simulink model "Manipulator2dof_SimMdl"  (R2026a)
settings: Solver=ode15s  StopTime=20  MaxStep=0.01
values from neighbouring files (symbols this model uses):
  d = 0.2    [Manipulator2dof_SimMdl_ini.m]
  T = 0.01    [Manipulator2dof_SimMdl_ini.m]
undefined symbols (not defined in the file or in its folder): l1, manip, X, Y, Z
libraries: sm_lib x16, nesl_utility x11, SignalEditorBlockLib x1
settings Model: Creator=Bender  LastModifiedBy=natte
settings SimscapeCC: SimscapeNominalValues="[{\"value\":\"1\",\"unit\":\"A\"},{\"value\":\"1\",\"unit\":\"bar\"},{\"value\":\"1\",\"unit\":\"cm^2\"},{\"value\":\"1\",\"unit\":\"cm^3/s\"},{\"value\":\"1\",\"unit\":\"kJ/kg\"},{\"value\":\"1\",\"unit\":\"kW\"},{\"value\":\"1\",\"unit\":\"l\"},{\"value\":\"1\",\"unit\":\"N\"},{\"value\":\"1\",\"unit\":\"N*m\"},{\"value\":\"1\",\"unit\":\"V\"}]"  SimscapeLogType=none  SimscapeLogDataHistory=5000.0

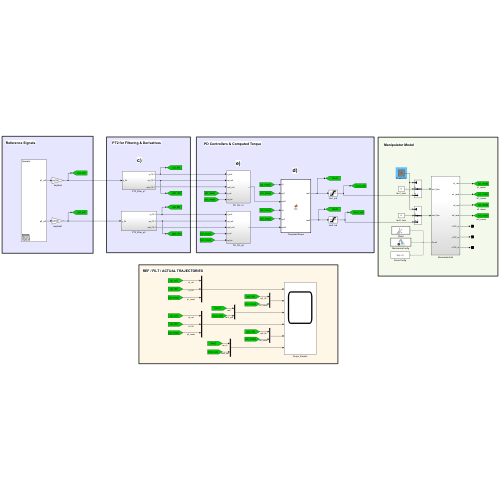
[thumbnail: Simulink's stored preview of the top-level diagram]
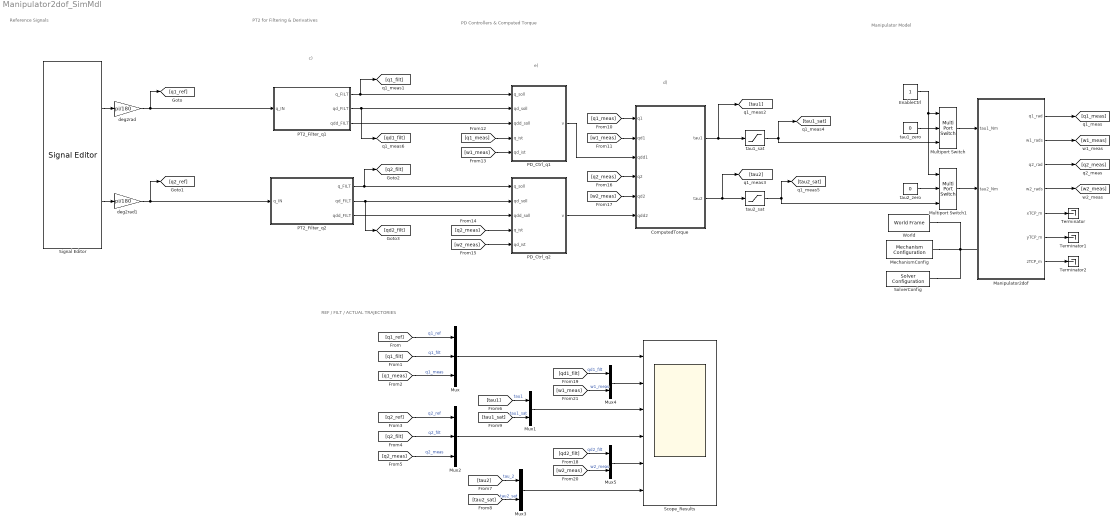
== system Manipulator2dof_SimMdl ==
  note: Reference Signals
  note: PT2 for Filtering & Derivatives
  note: PD Controllers & Computed Torque
  note: Manipulator Model
  note: REF / FILT / ACTUAL TRAJECTORIES
  note: d)
  note: c)
  note: e)
  ComputedTorque : MATLAB Function  TreatAsAtomicUnit=on
  EnableCtrl : Constant
  Manipulator2dof : Subsystem
  MechanismConfig : sm_lib/Utilities/Mechanism Configuration  UniformGravity=Constant  GravityVector=[0 0 -manip.g]  GravityVectorUnits=m/s^2  LinearizationDelta=0.001  JointModeTransitionNonlinearIterations=2
  Multiport Switch : MultiPortSwitch  DataPortOrder=Zero-based contiguous  Inputs=2  zeroidx=on  SaturateOnIntegerOverflow=off  InputSameDT=off
  Multiport Switch1 : MultiPortSwitch  DataPortOrder=Zero-based contiguous  Inputs=2  zeroidx=on  SaturateOnIntegerOverflow=off  InputSameDT=off
  Mux : Mux  Inputs=3
  Mux{1,3..5} (4 alike) : Mux  Inputs=2
  Mux2 : Mux  Inputs=3
  PD_Ctrl_q1 : Subsystem
  PD_Ctrl_q2 : Subsystem
  PT2_Filter_q1 : Subsystem
  PT2_Filter_q2 : Subsystem
  Scope_Results : Scope  NumInputPorts=6
      settings: ActiveDisplayYMinimum=-1  ActiveDisplayYMaximum=1
  Signal Editor : SignalEditorBlockLib/Signal Editor  FileName=Manipulator2dof_refSig.mat  ActiveScenario=Scenario  ActiveSignal=q1_ref  IsBus=off  OutputBusObjectStr=Bus: BusObject  SampleTime=0  ZeroCross=off  OutputAfterFinalValue=Setting to zero  Unit=inherit  PreserveSignalName=on  ApplySigPropsToAllScenarios=on  ApplySigPropsToAllSignals=off  SignalPropertySource=Dialog parameters
  SolverConfig : nesl_utility/Solver Configuration  PhysicalDomain=network_engine_domain  SubClassName=solver  LeftPortType=input  RightPortType=generic  Tones=[]  Harmonics=[]  SimulateNoise=off  Profile=off  UseLocalSampling=off  EnableSwitchedLinearOptims=on  FrequencyDomain=off  UseCCode=off  RelTol=0.001  AbsTol=0.001  MinStep=1e-09  ToWorkspace=off  RevertToSquareIcSolve=off  NumHomotopyIterations=100  PhasorMode=off  PhasorModeNumHarmonics=1  ConsistencySolver=NEWTON_XTOL_AFTER_FTOL  CanonicalOrdering=UNORDERED  OptimizeIntermediates=UNOPTIMIZED  IndexReductionMethod=DerivativeReplacement  DoDC=off  ResidualTolerance=1e-09  ConsistencyTolSource=GLOBAL  ConsistencyAbsTol=0.001  ConsistencyRelTol=0.001  ConsistencyTolFactor=0.001  UseLocalSolver=off  LocalSolverChoice=NE_BACKWARD_EULER_ADVANCER  ResolveIndetEquations=on  FunctionEvalNumThread=1  LocalSolverSampleTime=0.001  DoFixedCost=off  MaxNonlinIter=3  MaxModeIter=2  ComputeImpulses=off  ImpulseIterations=2  LinearAlgebra=auto  LinearAlgebraNumThread=0  EquationFormulation=NE_TIME_EF  DelaysMemoryBudget=1024  AutomaticFiltering=on  FilteringTimeConstant=0.001  PartitionStorageMethod=AS_NEEDED  PartitionMemoryBudget=1024  PartitionMethod=ROBUST  MultibodyUseLocalSolver=off  MultibodyLocalSolverChoice=ODE1  MultibodyLocalSolverSampleTime=0.001
  Terminator : Terminator
  Terminator1 : Terminator
  Terminator2 : Terminator
  World : sm_lib/Frames and Transforms/World Frame
  deg2rad : Gain  Gain=pi/180
  deg2rad1 : Gain  Gain=pi/180
  tau1_sat : Saturate  UpperLimit=manip.tau1_max  LowerLimit=-manip.tau1_max
  tau1_zero : Constant  Value=0
  tau2_sat : Saturate  UpperLimit=manip.tau2_max  LowerLimit=-manip.tau2_max
  tau2_zero : Constant  Value=0
  wires:
  Manipulator2dof/1(q1_rad) -> [q1_meas]
  Manipulator2dof/3(q2_rad) -> [q2_meas]
  Manipulator2dof/4(w2_rads) -> [w2_meas]
  tau1_sat/1 -> [tau1_sat], Multiport Switch/3
  Manipulator2dof/2(w1_rads) -> [w1_meas]
  tau2_sat/1 -> [tau2_sat], Multiport Switch1/3
  Mux/1 -> Scope_Results/1
  Signal Editor/1 -> deg2rad/1
  PT2_Filter_q1/1(q_FILT) -> [q1_filt], PD_Ctrl_q1/1(q_soll)
  PT2_Filter_q1/2(qd_FILT) -> [qd1_filt], PD_Ctrl_q1/2(qd_soll)
  PT2_Filter_q1/3(qdd_FILT) -> PD_Ctrl_q1/3(qdd_soll)
  deg2rad/1 -> PT2_Filter_q1/1(q_IN), [q1_ref]
  Signal Editor/2 -> deg2rad1/1
  Mux1/1 -> Scope_Results/3
  PT2_Filter_q2/1(q_FILT) -> PD_Ctrl_q2/1(q_soll), [q2_filt]
  PT2_Filter_q2/2(qd_FILT) -> [qd2_filt], PD_Ctrl_q2/2(qd_soll)
  PT2_Filter_q2/3(qdd_FILT) -> PD_Ctrl_q2/3(qdd_soll)
  deg2rad1/1 -> PT2_Filter_q2/1(q_IN), [q2_ref]
  Mux2/1 -> Scope_Results/4
  Mux3/1 -> Scope_Results/6
  [q1_meas] -> Mux/3  "q1_meas"
  [q1_filt] -> Mux/2  "q1_filt"
  [q1_ref] -> Mux/1  "q1_ref"
  [q2_ref] -> Mux2/1  "q2_ref"
  [q2_filt] -> Mux2/2  "q2_filt"
  [q2_meas] -> Mux2/3  "q2_meas"
  [tau1] -> Mux1/1  "tau1"
  [tau2] -> Mux3/1  "tau_2"
  [tau2_sat] -> Mux3/2  "tau2_sat"
  [tau1_sat] -> Mux1/2  "tau1_sat"
  ComputedTorque/1(tau1) -> tau1_sat/1, [tau1]
  ComputedTorque/2(tau2) -> tau2_sat/1, [tau2]
  PD_Ctrl_q1/1(v) -> ComputedTorque/3(qdd1)
  [q1_meas] -> ComputedTorque/1(q1)
  [w1_meas] -> ComputedTorque/2(qd1)
  [q1_meas] -> PD_Ctrl_q1/4(q_ist)
  [w1_meas] -> PD_Ctrl_q1/5(qd_ist)
  [q2_meas] -> PD_Ctrl_q2/4(q_ist)
  [w2_meas] -> PD_Ctrl_q2/5(qd_ist)
  PD_Ctrl_q2/1(v) -> ComputedTorque/6(qdd2)
  [q2_meas] -> ComputedTorque/4(q2)
  [w2_meas] -> ComputedTorque/5(qd2)
  Mux4/1 -> Scope_Results/2
  [qd1_filt] -> Mux4/1  "qd1_filt"
  Mux5/1 -> Scope_Results/5
  [qd2_filt] -> Mux5/1  "qd2_filt"
  [w2_meas] -> Mux5/2  "w2_meas"
  [w1_meas] -> Mux4/2  "w1_meas"
  Multiport Switch/1 -> Manipulator2dof/1(tau1_Nm)
  Multiport Switch1/1 -> Manipulator2dof/2(tau2_Nm)
  EnableCtrl/1 -> Multiport Switch1/1, Multiport Switch/1
  tau1_zero/1 -> Multiport Switch/2
  tau2_zero/1 -> Multiport Switch1/2
  Manipulator2dof/5(xTCP_m) -> Terminator/1
  Manipulator2dof/6(yTCP_m) -> Terminator1/1
  Manipulator2dof/7(zTCP_m) -> Terminator2/1
  connections:
  World/RConn1 -- MechanismConfig/RConn1 -- SolverConfig/RConn1 -- Manipulator2dof/LConn1

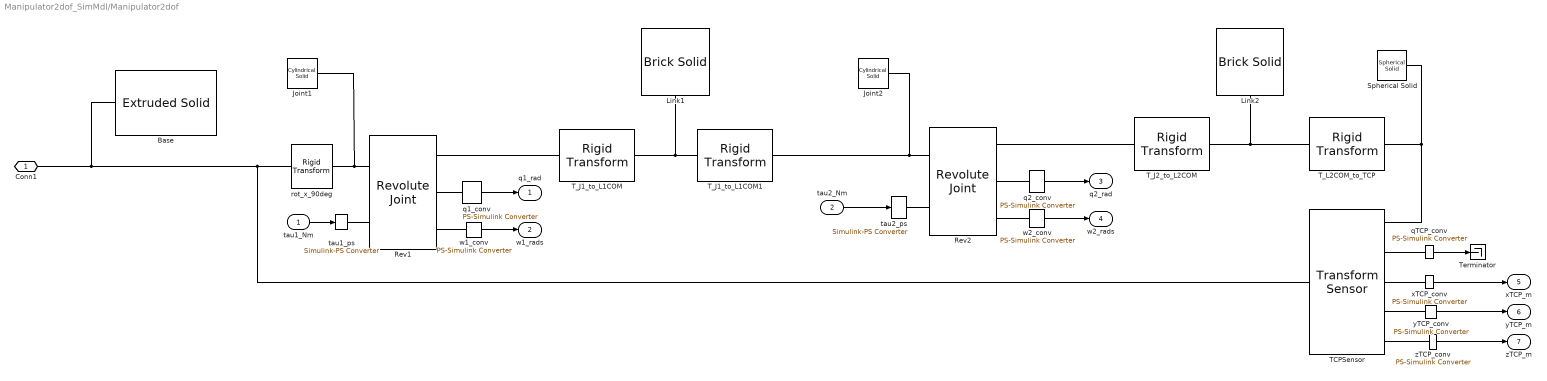
== system Manipulator2dof_SimMdl/Manipulator2dof ==
  tau1_Nm : Inport
  tau2_Nm : Inport  Port=2
  Base : sm_lib/Body Elements/Extruded Solid  ExtrusionType=Regular  PolygonNumSides=3  PolygonOuterRadius=0.2  PolygonOuterRadiusUnits=m  ExportEntireGeometry=off  ExtrusionCrossSection=[1 1; -1 1; -1 -1; 1 -1]  ExtrusionCrossSectionUnits=m  ExportConvexHullGeometry=off  ExtrusionLength=0.05  ExtrusionLengthUnits=m  InertiaType=PointMass  BasedOnType=Density  Density=1000  DensityUnits=kg/(m^3)  Mass=20  MassUnits=kg  CenterOfMass=[0 0 0]  CenterOfMassUnits=m  MomentsOfInertia=[10000 10000 10000]  MomentsOfInertiaUnits=kg*m^2  ProductsOfInertia=[10000 10000 10000]  ProductsOfInertiaUnits=kg*m^2  GraphicType=FromGeometry  MarkerShape=Sphere  MarkerSize=10  GraphicVisPropType=SimpleVisualProperties  GraphicDiffuseColor=[0.2 0.2 0.2]  GraphicOpacity=1  GraphicSpecularColor=[0.5 0.5 0.5 1.0]  GraphicAmbientColor=[0.15 0.15 0.15 1.0]  GraphicEmissiveColor=[0.0 0.0 0.0 1.0]  GraphicShininess=0  DoExposeReferenceFrame=off  SerializedFrames=<Frames><Frame><Id>Frame1</Id><Value><Name>F1</Name><Origin><Source>GeometricFeature</Source><FeatureName>side curve 2</FeatureName></Origin><PrimaryAxis><DefinedDirection>-Z</DefinedDirection><Source>GeometricFeature</Source><SourceDirection>+Z</SourceDirection><FeatureName>side surface 3</FeatureName></PrimaryAxis><SecondaryAxis><DefinedDirection>+X</DefinedDirection><Source>ReferenceFrame</Source><SourceDirection>+X</SourceDirection><FeatureName></FeatureName></SecondaryAxis></Value></Frame></Frames>
  Joint1 : sm_lib/Body Elements/Cylindrical Solid  CylinderRadius=0.05  CylinderRadiusUnits=m  CylinderLength=0.05  CylinderLengthUnits=m  ExportEntireGeometry=off  InertiaType=PointMass  BasedOnType=Density  Density=1000  DensityUnits=kg/m^3  Mass=0  MassUnits=kg  CenterOfMass=[0 0 0]  CenterOfMassUnits=m  MomentsOfInertia=[1 1 1]  MomentsOfInertiaUnits=kg*m^2  ProductsOfInertia=[0 0 0]  ProductsOfInertiaUnits=kg*m^2  GraphicType=FromGeometry  MarkerShape=Sphere  MarkerSize=10  GraphicVisPropType=SimpleVisualProperties  GraphicDiffuseColor=[0.7216 0.7216 0.7216]  GraphicOpacity=1  GraphicSpecularColor=[0.5 0.5 0.5 1.0]  GraphicAmbientColor=[0.15 0.15 0.15 1.0]  GraphicEmissiveColor=[0.0 0.0 0.0 1.0]  GraphicShininess=75  DoExposeReferenceFrame=on  SerializedFrames=<Frames/>
  Joint2 : sm_lib/Body Elements/Cylindrical Solid  CylinderRadius=0.05  CylinderRadiusUnits=m  CylinderLength=0.05  CylinderLengthUnits=m  ExportEntireGeometry=off  InertiaType=PointMass  BasedOnType=Density  Density=1000  DensityUnits=kg/m^3  Mass=manip.m1plant  MassUnits=kg  CenterOfMass=[0 0 0]  CenterOfMassUnits=m  MomentsOfInertia=[1 1 1]  MomentsOfInertiaUnits=kg*m^2  ProductsOfInertia=[0 0 0]  ProductsOfInertiaUnits=kg*m^2  GraphicType=FromGeometry  MarkerShape=Sphere  MarkerSize=10  GraphicVisPropType=SimpleVisualProperties  GraphicDiffuseColor=[0.7216 0.7216 0.7216]  GraphicOpacity=1  GraphicSpecularColor=[0.5 0.5 0.5 1.0]  GraphicAmbientColor=[0.15 0.15 0.15 1.0]  GraphicEmissiveColor=[0.0 0.0 0.0 1.0]  GraphicShininess=75  DoExposeReferenceFrame=on  SerializedFrames=<Frames/>
  Link1 : sm_lib/Body Elements/Brick Solid  BrickDimensions=[manip.l1 manip.linkWidth manip.linkThickness]  BrickDimensionsUnits=m  ExportEntireGeometry=off  InertiaType=PointMass  BasedOnType=Density  Density=rho1  DensityUnits=kg/m^3  Mass=0  MassUnits=kg  CenterOfMass=[0 0 0]  CenterOfMassUnits=m  MomentsOfInertia=[1 1 1]  MomentsOfInertiaUnits=kg*m^2  ProductsOfInertia=[0 0 0]  ProductsOfInertiaUnits=kg*m^2  GraphicType=FromGeometry  MarkerShape=Sphere  MarkerSize=10  GraphicVisPropType=SimpleVisualProperties  GraphicDiffuseColor=[0.5 0.5 0.5]  GraphicOpacity=1  GraphicSpecularColor=[0.5 0.5 0.5 1.0]  GraphicAmbientColor=[0.15 0.15 0.15 1.0]  GraphicEmissiveColor=[0.0 0.0 0.0 1.0]  GraphicShininess=75  DoExposeReferenceFrame=on  SerializedFrames=<Frames/>
  Link2 : sm_lib/Body Elements/Brick Solid  BrickDimensions=[manip.l2 manip.linkWidth manip.linkThickness]  BrickDimensionsUnits=m  ExportEntireGeometry=off  InertiaType=PointMass  BasedOnType=Density  Density=rho2  DensityUnits=kg/m^3  Mass=0  MassUnits=kg  CenterOfMass=[0 0 0]  CenterOfMassUnits=m  MomentsOfInertia=[1 1 1]  MomentsOfInertiaUnits=kg*m^2  ProductsOfInertia=[0 0 0]  ProductsOfInertiaUnits=kg*m^2  GraphicType=FromGeometry  MarkerShape=Sphere  MarkerSize=10  GraphicVisPropType=SimpleVisualProperties  GraphicDiffuseColor=[0.5 0.5 0.5]  GraphicOpacity=1  GraphicSpecularColor=[0.5 0.5 0.5 1.0]  GraphicAmbientColor=[0.15 0.15 0.15 1.0]  GraphicEmissiveColor=[0.0 0.0 0.0 1.0]  GraphicShininess=75  DoExposeReferenceFrame=on  SerializedFrames=<Frames/>
  Rev1 : sm_lib/Joints/Revolute Joint  JointMode=Normal  CompositeWrenchDir=FollowerOnBase  CompositeWrenchFrame=BaseFrame  SenseConstraintForce=off  SenseConstraintTorque=off  SenseTotalForce=off  SenseTotalTorque=off  PositionTargetSpecify=off  PositionTargetPriority=High  PositionTargetValue=0  PositionTargetValueUnits=deg  VelocityTargetSpecify=off  VelocityTargetPriority=High  VelocityTargetValue=0  VelocityTargetValueUnits=deg/s  EquilibriumPosition=0  EquilibriumPositionUnits=deg  SpringStiffness=0  SpringStiffnessUnits=N*m/deg  DampingCoefficient=0  DampingCoefficientUnits=N*m/(deg/s)  LowerLimitSpecify=off  LowerLimitBound=manip.theta1_min  LowerLimitBoundUnits=deg  LowerLimitStiffness=manip.kLimit  LowerLimitStiffnessUnits=N*m/deg  LowerLimitDamping=manip.dLimit  LowerLimitDampingUnits=N*m/(deg/s)  LowerLimitTransitionRegionWidth=manip.limitTransition  LowerLimitTransitionRegionWidthUnits=deg  UpperLimitSpecify=off  UpperLimitBound=manip.theta1_max  UpperLimitBoundUnits=deg  UpperLimitStiffness=manip.kLimit  UpperLimitStiffnessUnits=N*m/deg  UpperLimitDamping=manip.dLimit  UpperLimitDampingUnits=N*m/(deg/s)  UpperLimitTransitionRegionWidth=manip.limitTransition  UpperLimitTransitionRegionWidthUnits=deg  TorqueActuationMode=InputTorque  MotionActuationMode=ComputedMotion  SensePosition=on  SenseVelocity=on  SenseAcceleration=off  SenseTorqueForce=off  SenseLowerLimitTorqueForce=off  SenseUpperLimitTorqueForce=off
  Rev2 : sm_lib/Joints/Revolute Joint  JointMode=Normal  CompositeWrenchDir=FollowerOnBase  CompositeWrenchFrame=BaseFrame  SenseConstraintForce=off  SenseConstraintTorque=off  SenseTotalForce=off  SenseTotalTorque=off  PositionTargetSpecify=off  PositionTargetPriority=High  PositionTargetValue=0  PositionTargetValueUnits=deg  VelocityTargetSpecify=off  VelocityTargetPriority=High  VelocityTargetValue=0  VelocityTargetValueUnits=deg/s  EquilibriumPosition=0  EquilibriumPositionUnits=deg  SpringStiffness=0  SpringStiffnessUnits=N*m/deg  DampingCoefficient=0  DampingCoefficientUnits=N*m/(deg/s)  LowerLimitSpecify=off  LowerLimitBound=manip.theta2_min  LowerLimitBoundUnits=deg  LowerLimitStiffness=manip.kLimit  LowerLimitStiffnessUnits=N*m/deg  LowerLimitDamping=manip.dLimit  LowerLimitDampingUnits=N*m/(deg/s)  LowerLimitTransitionRegionWidth=manip.limitTransition  LowerLimitTransitionRegionWidthUnits=deg  UpperLimitSpecify=off  UpperLimitBound=manip.theta2_max  UpperLimitBoundUnits=deg  UpperLimitStiffness=manip.kLimit  UpperLimitStiffnessUnits=N*m/deg  UpperLimitDamping=manip.dLimit  UpperLimitDampingUnits=N*m/(deg/s)  UpperLimitTransitionRegionWidth=manip.limitTransition  UpperLimitTransitionRegionWidthUnits=deg  TorqueActuationMode=InputTorque  MotionActuationMode=ComputedMotion  SensePosition=on  SenseVelocity=on  SenseAcceleration=off  SenseTorqueForce=off  SenseLowerLimitTorqueForce=off  SenseUpperLimitTorqueForce=off
  Spherical Solid : sm_lib/Body Elements/Spherical Solid  SphereRadius=0.05  SphereRadiusUnits=m  ExportEntireGeometry=off  InertiaType=PointMass  BasedOnType=Density  Density=1000  DensityUnits=kg/m^3  Mass=manip.m2plant  MassUnits=kg  CenterOfMass=[0 0 0]  CenterOfMassUnits=m  MomentsOfInertia=[1 1 1]  MomentsOfInertiaUnits=kg*m^2  ProductsOfInertia=[0 0 0]  ProductsOfInertiaUnits=kg*m^2  GraphicType=FromGeometry  MarkerShape=Sphere  MarkerSize=10  GraphicVisPropType=SimpleVisualProperties  GraphicDiffuseColor=[0 0 1]  GraphicOpacity=1  GraphicSpecularColor=[0.5 0.5 0.5 1.0]  GraphicAmbientColor=[0.15 0.15 0.15 1.0]  GraphicEmissiveColor=[0.0 0.0 0.0 1.0]  GraphicShininess=75  DoExposeReferenceFrame=on  SerializedFrames=<Frames/>
  TCPSensor : sm_lib/Frames and Transforms/Transform Sensor  MeasurementFrame=World  RotationSequence=XYX  SenseAngle=off  SenseAxis=off  SenseQ=on  SenseR=off  SenseRotationSequence=off  SenseOmegaX=off  SenseOmegaY=off  SenseOmegaZ=off  SenseOmega=off  SenseQDot=off  SenseRDot=off  SenseRotationSequenceDot=off  SenseAlphaX=off  SenseAlphaY=off  SenseAlphaZ=off  SenseAlpha=off  SenseQDDot=off  SenseRDDot=off  SenseX=on  SenseY=on  SenseZ=on  SenseXYZ=off  SenseRad=off  SenseAzim=off  SenseDist=off  SenseInc=off  SenseXDot=off  SenseYDot=off  SenseZDot=off  SenseXYZDot=off  SenseRadDot=off  SenseAzimDot=off  SenseDistDot=off  SenseIncDot=off  SenseXDDot=off  SenseYDDot=off  SenseZDDot=off  SenseXYZDDot=off  SenseRadDDot=off  SenseAzimDDot=off  SenseDistDDot=off  SenseIncDDot=off
  T_J1_to_L1COM : sm_lib/Frames and Transforms/Rigid Transform  RotationMethod=None  FollAlignAxisA=+X  BaseAlignAxisA=+Y  FollAlignAxisB=+Y  BaseAlignAxisB=+Z  RotationStandardAxis=+Z  RotationAngle=0  RotationAngleUnits=deg  RotationArbitraryAxis=[0 0 1]  RotationSequenceAxes=FollowerAxes  RotationSequence=XYX  RotationSequenceAngles=[0 0 0]  RotationSequenceAnglesUnits=deg  RotationMatrix=[1 0 0;0 1 0;0 0 1]  Quaternion=[1 0 0 0]  TranslationMethod=StandardAxis  TranslationCartesianOffset=[0 0 0]  TranslationCartesianOffsetUnits=m  TranslationStandardAxis=+X  TranslationStandardOffset=manip.l1/2  TranslationStandardOffsetUnits=m  TranslationROffset=0  TranslationROffsetUnits=m  TranslationThetaOffset=0  TranslationThetaOffsetUnits=deg  TranslationZOffset=0  TranslationZOffsetUnits=m
  T_J1_to_L1COM1 : sm_lib/Frames and Transforms/Rigid Transform  RotationMethod=None  FollAlignAxisA=+X  BaseAlignAxisA=+Y  FollAlignAxisB=+Y  BaseAlignAxisB=+Z  RotationStandardAxis=+Z  RotationAngle=0  RotationAngleUnits=deg  RotationArbitraryAxis=[0 0 1]  RotationSequenceAxes=FollowerAxes  RotationSequence=XYX  RotationSequenceAngles=[0 0 0]  RotationSequenceAnglesUnits=deg  RotationMatrix=[1 0 0;0 1 0;0 0 1]  Quaternion=[1 0 0 0]  TranslationMethod=StandardAxis  TranslationCartesianOffset=[0 0 0]  TranslationCartesianOffsetUnits=m  TranslationStandardAxis=+X  TranslationStandardOffset=manip.l1/2  TranslationStandardOffsetUnits=m  TranslationROffset=0  TranslationROffsetUnits=m  TranslationThetaOffset=0  TranslationThetaOffsetUnits=deg  TranslationZOffset=0  TranslationZOffsetUnits=m
  T_J2_to_L2COM : sm_lib/Frames and Transforms/Rigid Transform  RotationMethod=None  FollAlignAxisA=+X  BaseAlignAxisA=+Y  FollAlignAxisB=+Y  BaseAlignAxisB=+Z  RotationStandardAxis=+Z  RotationAngle=0  RotationAngleUnits=deg  RotationArbitraryAxis=[0 0 1]  RotationSequenceAxes=FollowerAxes  RotationSequence=XYX  RotationSequenceAngles=[0 0 0]  RotationSequenceAnglesUnits=deg  RotationMatrix=[1 0 0;0 1 0;0 0 1]  Quaternion=[1 0 0 0]  TranslationMethod=StandardAxis  TranslationCartesianOffset=[0 0 0]  TranslationCartesianOffsetUnits=m  TranslationStandardAxis=+X  TranslationStandardOffset=manip.l2/2  TranslationStandardOffsetUnits=m  TranslationROffset=0  TranslationROffsetUnits=m  TranslationThetaOffset=0  TranslationThetaOffsetUnits=deg  TranslationZOffset=0  TranslationZOffsetUnits=m
  T_L2COM_to_TCP : sm_lib/Frames and Transforms/Rigid Transform  RotationMethod=None  FollAlignAxisA=+X  BaseAlignAxisA=+Y  FollAlignAxisB=+Y  BaseAlignAxisB=+Z  RotationStandardAxis=+Z  RotationAngle=0  RotationAngleUnits=deg  RotationArbitraryAxis=[0 0 1]  RotationSequenceAxes=FollowerAxes  RotationSequence=XYX  RotationSequenceAngles=[0 0 0]  RotationSequenceAnglesUnits=deg  RotationMatrix=[1 0 0;0 1 0;0 0 1]  Quaternion=[1 0 0 0]  TranslationMethod=StandardAxis  TranslationCartesianOffset=[0 0 0]  TranslationCartesianOffsetUnits=m  TranslationStandardAxis=+X  TranslationStandardOffset=manip.l2/2  TranslationStandardOffsetUnits=m  TranslationROffset=0  TranslationROffsetUnits=m  TranslationThetaOffset=0  TranslationThetaOffsetUnits=deg  TranslationZOffset=0  TranslationZOffsetUnits=m
  Terminator : Terminator
  q1_conv : nesl_utility/PS-Simulink Converter  PhysicalDomain=network_engine_domain  SubClassName=ps_output  LeftPortType=input  RightPortType=output  PseudoPeriodic=off  Frequencies=[]  VectorFormat=inherit  Unit=rad  AffineConversion=off
  q2_conv : nesl_utility/PS-Simulink Converter  PhysicalDomain=network_engine_domain  SubClassName=ps_output  LeftPortType=input  RightPortType=output  PseudoPeriodic=off  Frequencies=[]  VectorFormat=inherit  Unit=rad  AffineConversion=off
  qTCP_conv : nesl_utility/PS-Simulink Converter  PhysicalDomain=network_engine_domain  SubClassName=ps_output  LeftPortType=input  RightPortType=output  PseudoPeriodic=off  Frequencies=[]  VectorFormat=inherit  Unit=1  AffineConversion=off
  rot_x_90deg : sm_lib/Frames and Transforms/Rigid Transform  RotationMethod=StandardAxis  FollAlignAxisA=+X  BaseAlignAxisA=+Y  FollAlignAxisB=+Y  BaseAlignAxisB=+Z  RotationStandardAxis=+X  RotationAngle=90  RotationAngleUnits=deg  RotationArbitraryAxis=[0 0 1]  RotationSequenceAxes=FollowerAxes  RotationSequence=XYX  RotationSequenceAngles=[0 0 0]  RotationSequenceAnglesUnits=deg  RotationMatrix=[1 0 0;0 1 0;0 0 1]  Quaternion=[1 0 0 0]  TranslationMethod=None  TranslationCartesianOffset=[0 0 0]  TranslationCartesianOffsetUnits=m  TranslationStandardAxis=+X  TranslationStandardOffset=l1/2  TranslationStandardOffsetUnits=m  TranslationROffset=0  TranslationROffsetUnits=m  TranslationThetaOffset=0  TranslationThetaOffsetUnits=deg  TranslationZOffset=0  TranslationZOffsetUnits=m
  tau1_ps : nesl_utility/Simulink-PS Converter  PhysicalDomain=network_engine_domain  SubClassName=ps_input  LeftPortType=input  RightPortType=output  PseudoPeriodic=off  Frequencies=[]  NoiseDistribution=none  NoiseParameters=[]  Unit=N*m  AffineConversion=off  FilteringAndDerivatives=provide  SimscapeFilterOrder=1  InputFilterTimeConstant=0.001  UdotUserProvided=0
  tau2_ps : nesl_utility/Simulink-PS Converter  PhysicalDomain=network_engine_domain  SubClassName=ps_input  LeftPortType=input  RightPortType=output  PseudoPeriodic=off  Frequencies=[]  NoiseDistribution=none  NoiseParameters=[]  Unit=N*m  AffineConversion=off  FilteringAndDerivatives=provide  SimscapeFilterOrder=1  InputFilterTimeConstant=0.001  UdotUserProvided=0
  w1_conv : nesl_utility/PS-Simulink Converter  PhysicalDomain=network_engine_domain  SubClassName=ps_output  LeftPortType=input  RightPortType=output  PseudoPeriodic=off  Frequencies=[]  VectorFormat=inherit  Unit=rad/s  AffineConversion=off
  w2_conv : nesl_utility/PS-Simulink Converter  PhysicalDomain=network_engine_domain  SubClassName=ps_output  LeftPortType=input  RightPortType=output  PseudoPeriodic=off  Frequencies=[]  VectorFormat=inherit  Unit=rad/s  AffineConversion=off
  xTCP_conv : nesl_utility/PS-Simulink Converter  PhysicalDomain=network_engine_domain  SubClassName=ps_output  LeftPortType=input  RightPortType=output  PseudoPeriodic=off  Frequencies=[]  VectorFormat=inherit  Unit=m  AffineConversion=off
  yTCP_conv : nesl_utility/PS-Simulink Converter  PhysicalDomain=network_engine_domain  SubClassName=ps_output  LeftPortType=input  RightPortType=output  PseudoPeriodic=off  Frequencies=[]  VectorFormat=inherit  Unit=m  AffineConversion=off
  zTCP_conv : nesl_utility/PS-Simulink Converter  PhysicalDomain=network_engine_domain  SubClassName=ps_output  LeftPortType=input  RightPortType=output  PseudoPeriodic=off  Frequencies=[]  VectorFormat=inherit  Unit=m  AffineConversion=off
  Conn1 : PMIOPort  Side=Left
  q1_rad : Outport
  w1_rads : Outport  Port=2
  q2_rad : Outport  Port=3
  w2_rads : Outport  Port=4
  xTCP_m : Outport  Port=5
  yTCP_m : Outport  Port=6
  zTCP_m : Outport  Port=7
  wires:
  zTCP_conv/1 -> zTCP_m/1
  q1_conv/1 -> q1_rad/1
  yTCP_conv/1 -> yTCP_m/1
  xTCP_conv/1 -> xTCP_m/1
  tau2_Nm/1 -> tau2_ps/1
  w2_conv/1 -> w2_rads/1
  w1_conv/1 -> w1_rads/1
  q2_conv/1 -> q2_rad/1
  tau1_Nm/1 -> tau1_ps/1
  qTCP_conv/1 -> Terminator/1
  connections:
  Rev1/RConn2 -- q1_conv/LConn1
  tau1_ps/RConn1 -- Rev1/LConn2
  T_J1_to_L1COM/RConn1 -- T_J1_to_L1COM1/LConn1 -- Link1/RConn1
  T_L2COM_to_TCP/RConn1 -- TCPSensor/RConn1 -- Spherical Solid/RConn1
  T_J2_to_L2COM/RConn1 -- T_L2COM_to_TCP/LConn1 -- Link2/RConn1
  tau2_ps/RConn1 -- Rev2/LConn2
  TCPSensor/RConn4 -- yTCP_conv/LConn1
  TCPSensor/RConn5 -- zTCP_conv/LConn1
  xTCP_conv/LConn1 -- TCPSensor/RConn3
  TCPSensor/RConn2 -- qTCP_conv/LConn1
  Rev2/RConn3 -- w2_conv/LConn1
  Rev1/RConn3 -- w1_conv/LConn1
  Rev2/RConn1 -- T_J2_to_L2COM/LConn1
  Rev1/RConn1 -- T_J1_to_L1COM/LConn1
  Joint2/RConn1 -- T_J1_to_L1COM1/RConn1 -- Rev2/LConn1
  Rev2/RConn2 -- q2_conv/LConn1
  rot_x_90deg/RConn1 -- Joint1/RConn1 -- Rev1/LConn1
  Conn1/RConn1 -- Base/LConn1 -- TCPSensor/LConn1 -- rot_x_90deg/LConn1

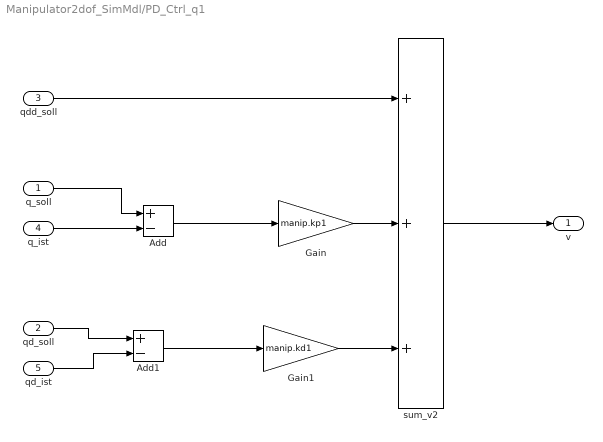
== system Manipulator2dof_SimMdl/PD_Ctrl_q1 ==
  q_soll : Inport
  qd_soll : Inport  Port=2
  qdd_soll : Inport  Port=3
  q_ist : Inport  Port=4
  qd_ist : Inport  Port=5
  Add : Sum  Inputs=+-
  Add1 : Sum  Inputs=+-
  Gain : Gain  Gain=manip.kp1
  Gain1 : Gain  Gain=manip.kd1
  sum_v2 : Sum  Inputs=+++
  v : Outport
  wires:
  qdd_soll/1 -> sum_v2/1
  sum_v2/1 -> v/1
  q_ist/1 -> Add/2
  q_soll/1 -> Add/1
  Gain/1 -> sum_v2/2
  Add/1 -> Gain/1
  qd_ist/1 -> Add1/2
  qd_soll/1 -> Add1/1
  Add1/1 -> Gain1/1
  Gain1/1 -> sum_v2/3

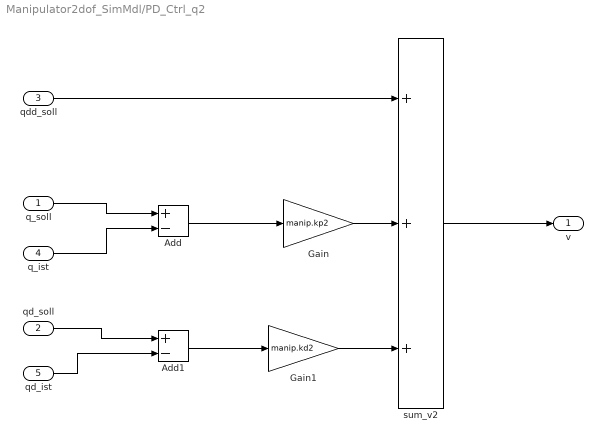
== system Manipulator2dof_SimMdl/PD_Ctrl_q2 ==
  q_soll : Inport
  qd_soll : Inport  Port=2
  qdd_soll : Inport  Port=3
  q_ist : Inport  Port=4
  qd_ist : Inport  Port=5
  Add : Sum  Inputs=+-
  Add1 : Sum  Inputs=+-
  Gain : Gain  Gain=manip.kp2
  Gain1 : Gain  Gain=manip.kd2
  sum_v2 : Sum  Inputs=+++
  v : Outport
  wires:
  sum_v2/1 -> v/1
  qdd_soll/1 -> sum_v2/1
  q_soll/1 -> Add/1
  q_ist/1 -> Add/2
  Add/1 -> Gain/1
  Gain/1 -> sum_v2/2
  qd_soll/1 -> Add1/1
  qd_ist/1 -> Add1/2
  Add1/1 -> Gain1/1
  Gain1/1 -> sum_v2/3

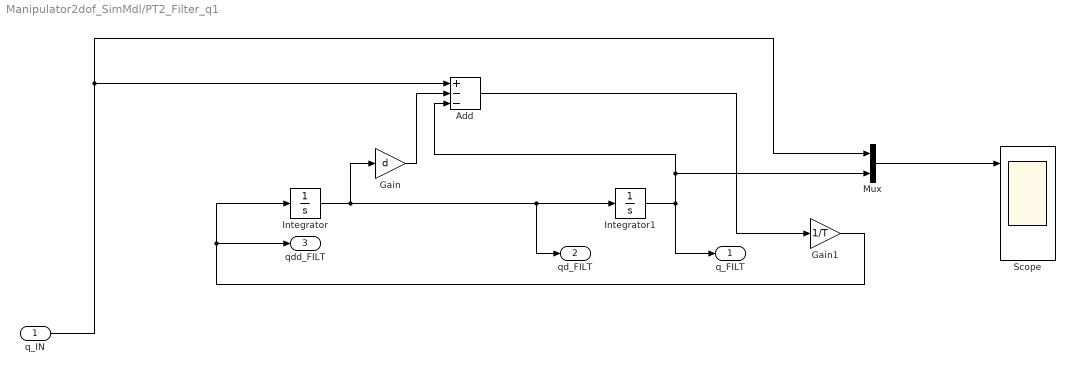
== system Manipulator2dof_SimMdl/PT2_Filter_q1 ==
  q_IN : Inport
  Add : Sum  Inputs=+--
  Gain : Gain  Gain=d
  Gain1 : Gain  Gain=1/T
  Integrator : Integrator
  Integrator1 : Integrator
  Mux : Mux  Inputs=2
  Scope : Scope  NumInputPorts=3
      settings: ActiveDisplayYMinimum=-0.64815234126413657  ActiveDisplayYMaximum=2.454504090692895
  q_FILT : Outport
  qd_FILT : Outport  Port=2
  qdd_FILT : Outport  Port=3
  wires:
  Mux/1 -> Scope/1
  Integrator/1 -> Gain/1, qd_FILT/1, Integrator1/1
  Integrator1/1 -> Mux/2, Add/3, q_FILT/1
  Gain1/1 -> Integrator/1, qdd_FILT/1
  q_IN/1 -> Add/1, Mux/1
  Gain/1 -> Add/2
  Add/1 -> Gain1/1

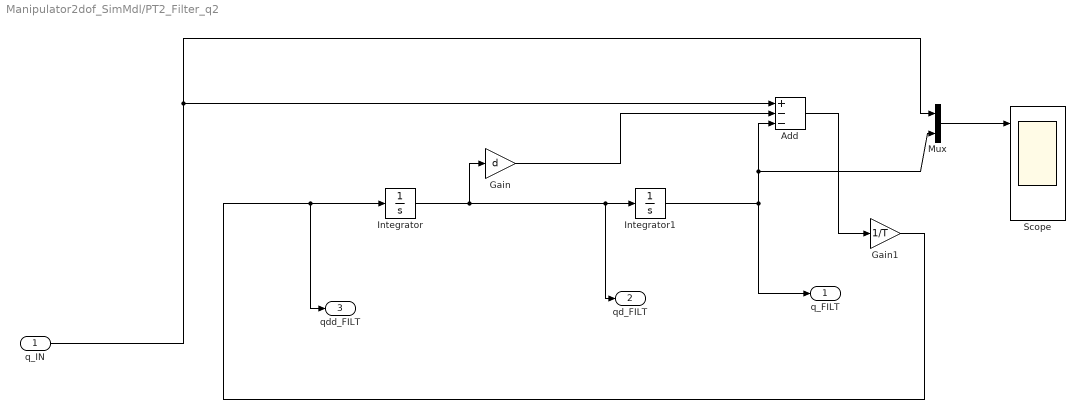
== system Manipulator2dof_SimMdl/PT2_Filter_q2 ==
  q_IN : Inport
  Add : Sum  Inputs=+--
  Gain : Gain  Gain=d
  Gain1 : Gain  Gain=1/T
  Integrator : Integrator
  Integrator1 : Integrator
  Mux : Mux  Inputs=2
  Scope : Scope  NumInputPorts=3
      settings: ActiveDisplayYMinimum=-0.06545171809593528  ActiveDisplayYMaximum=0.58905185398424742
  q_FILT : Outport
  qd_FILT : Outport  Port=2
  qdd_FILT : Outport  Port=3
  wires:
  Mux/1 -> Scope/1
  Gain1/1 -> Integrator/1, qdd_FILT/1
  Integrator/1 -> Gain/1, qd_FILT/1, Integrator1/1
  Integrator1/1 -> Add/3, Mux/2, q_FILT/1
  q_IN/1 -> Mux/1, Add/1
  Gain/1 -> Add/2
  Add/1 -> Gain1/1

== matlab function Manipulator2dof_SimMdl/ComputedTorque ==
  data: q1 input; tau1 output; qd1 input; qdd1 input; q2 input; qd2 input; qdd2 input; tau2 output; manip parameter
function [tau1,tau2] = fcn(q1,qd1,qdd1,q2,qd2,qdd2, manip)
% Computed Torque approach: 
% Drive Torques tau1 and tau2 are calculated via Manipulator-Dynamic:
% M(q)qdd + C(q,qd)*qd + g(q) = tau

m1 = manip.m1;
m2 = manip.m2;
l1 = manip.l1;
l2 = manip.l2;
g  = manip.g; % earth acceleration g [m/s^2]

% ------------- Exercise 1.2 d) ------------------------------
% elements of inertia matrix M(q)
M11 = (m1 + m2)*l1^2 + m2*l2^2 + 2*m2*l1*l2*cos(q2);
M12 = m2*l2^2 + m2*l1*l2*cos(q2);
M21 = m2*l2^2 + m2*l1*l2*cos(q2);
M22 = m2*l2^2;

% Coriolis and centrifugal forces (vector components)
C1 = -m2*l1*l2*sin(q2)*(2*qd1*qd2 + qd2^2);
C2 =  m2*l1*l2*(qd1^2)*sin(q2);

% Gravitational power (Vector-components)
g1 = (m1 + m2)*g*l1*cos(q1) + m2*g*l2*cos(q1 + q2);
g2 =  m2*g*l2*cos(q1 + q2);

% create vectors and matrix
M   = [M11, M12; 
       M21, M22];
qdd = [qdd1; qdd2];

C   = [C1; C2];
qd  = [qd1; qd2];

g_vec = [g1; g2];

% calculate Drive Torque tau = M(q)*qdd + C(q,qd) + g(q)
tau = M*qdd + C + g_vec;

% assert to output variables
tau1 = tau(1);
tau2 = tau(2);
